simulink subsystem "Subsys_Conv_Ctrl_measurement_transformations"  (R2022b)
settings: Solver=VariableStepAuto  StartTime=0.0  StopTime=10.0  RelTol=1e-3
model mask{S_n=2e6, f_n=50, V_n_phph=690, V_n_grid_phph=20e3, V_n_dc=1380, meas_signals=0, meas_noise_filter=1, f_cutoff_lowpass=2500, posseq_calc=0, f_cutoff_posseq=20, prot_variant=1, v_dc_max=1.2, v_ac_max=1.1, t_ac_max=0.1, v_ac_maxmax=1.25, t_ac_maxmax=0.1, v_ac_min=0.8, t_ac_min=3, v_ac_minmin=0.45, t_ac_minmin=0.3, f_ac_max=51.5, t_f_ac_max=0.1, f_ac_maxmax=52.5, t_f_ac_maxmax=10, f_ac_min=47.5, t_f_ac_min=0.1, i_ac_max=1.25, T_s_ctrl=1e-3, T_s_PWM_meas=1e-4, datatype='double'}
  mask prompts: S_n "Nominal power [VA]"; f_n "Nominal frequency [Hz]"; V_n_phph "Nominal converter voltage (rms, phase-to-phase) [V]"; V_n_grid_phph "Nominal grid voltage (rms, phase-to-phase) [V]"; V_n_dc "Nominal DC-link voltage [V]"; meas_signals "Measured signals (0 = all signals (tDMSquared simulation), 1 = reduced signals (imperix hardware))"; meas_noise_filter "Low-pass to filter measurement noise (1 = enabled, 0 = disabled)"; f_cutoff_lowpass "Cutoff-frequency of low pass filter (measurement noise) [Hz]"; posseq_calc "Positive sequence calculation (0 = DDSRF, 1 = low pass filter)"; f_cutoff_posseq "Cutoff-frequency of low pass filter (positive sequence calculation) [Hz]"; prot_variant "Protection Variant (1 = hardware protection, 2 = tDMSquared warnings only, 3 = deactivated)"; v_dc_max "Maximum DC-link voltage [% nom. value]"; v_ac_max "Lower Maximum AC voltage [% nom. value]"; t_ac_max "Lower Maximum AC voltage timing [s]"; v_ac_maxmax "Upper Maximum AC voltage [% nom. value]"; t_ac_maxmax "Upper Maximum AC voltage timing [s]"; v_ac_min "Upper Minimum AC voltage [% nom. value]"; t_ac_min "Upper Minimum AC voltage timing [s]"; v_ac_minmin "Lower Minimum AC voltage [% nom. value]"; t_ac_minmin "Lower Minimum AC voltage timing [s]"; f_ac_max "Maximum AC frequency [Hz]"; t_f_ac_max "Maximum AC frequency timing [s]"; f_ac_maxmax "Upper Maximum AC frequency [Hz]"; t_f_ac_maxmax "Upper Maximum AC frequency timing [s]"; f_ac_min "Minimum AC frequency [Hz]"; t_f_ac_min "Minimum AC frequency timing [s]"; i_ac_max "Maximum AC current [% nom. value]"; T_s_ctrl "Controller sample time [s]"; T_s_PWM_meas "PWM and measurements sample time [s]"; datatype "Signal data type"
undefined symbols (not defined in the file): alpha_meas_LPF, alpha_posseq_LPF, den_HPF, num_HPF
libraries: eeTransforms x18
settings Model: Creator=winkens  LastModifiedBy=pc236admin
settings SolverCC: AlgebraicLoopSolver=TrustRegion
settings DebuggingCC: UnconnectedInputMsg=warning  UnconnectedOutputMsg=warning  UnconnectedLineMsg=warning  SFMachineParentedDataDiag=warning
settings ModelReferenceCC: EnableRefExpFcnMdlSchedulingChecks=on
settings RTWCC: DLArmComputeVersion=19.05

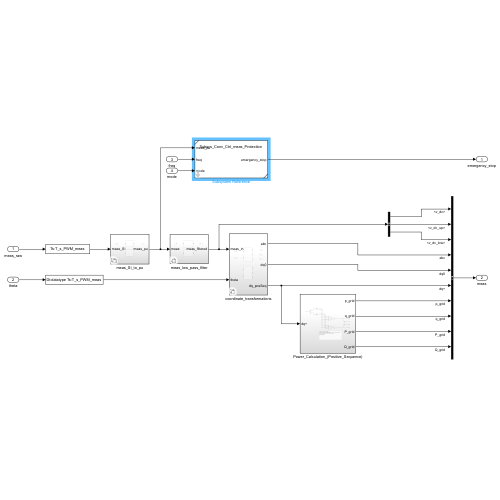
[thumbnail: Simulink's stored preview of the top-level diagram]
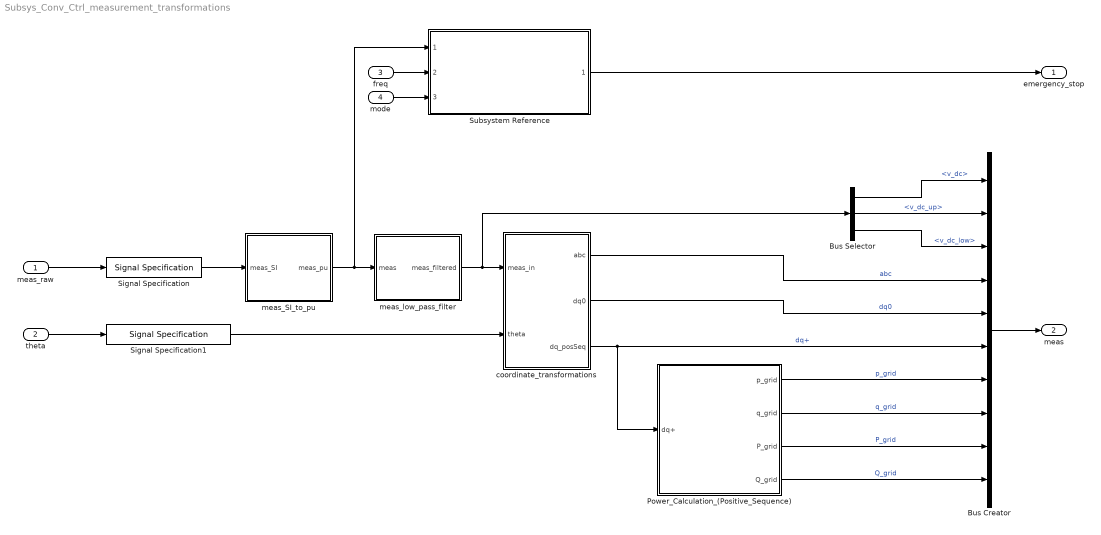
== system Subsys_Conv_Ctrl_measurement_transformations ==
  meas_raw : Inport
  theta : Inport  Port=2
  freq : Inport  Port=3
  mode : Inport  Port=4
  Bus Creator : BusCreator  Inputs=10
  Bus Selector : BusSelector  OutputSignals=v_dc,v_dc_up,v_dc_low
  Power_Calculation_(Positive_Sequence) : Subsystem
  Signal Specification : SignalSpecification  SampleTime=T_s_PWM_meas
  Signal Specification1 : SignalSpecification  OutDataTypeStr=datatype  SampleTime=T_s_PWM_meas
  Subsystem Reference : Subsystem  ReferencedSubsystem=Subsys_Conv_Ctrl_meas_Protection  prot_variant=prot_variant  f_n=f_n  meas_signals=meas_signals  v_n_dc=1  v_dc_max=v_dc_max  v_ac_max=v_ac_max  t_ac_max=t_ac_max  v_ac_maxmax=v_ac_maxmax  t_ac_maxmax=t_ac_maxmax  v_ac_min=v_ac_min  t_ac_min=t_ac_min  v_ac_minmin=v_ac_minmin  t_ac_minmin=t_ac_minmin  f_ac_max=f_ac_max  t_f_ac_max=t_f_ac_max  f_ac_maxmax=f_ac_maxmax  t_f_ac_maxmax=t_f_ac_maxmax  f_ac_min=f_ac_min  t_f_ac_min=t_f_ac_min  i_ac_max=i_ac_max  T_s=T_s_PWM_meas
  coordinate_transformations : Subsystem  Variant=on  VariantControl=Choice
  meas_SI_to_pu : Subsystem  Variant=on  VariantControl=Choice
  meas_low_pass_filter : Subsystem  Variant=on  VariantControl=Choice
  emergency_stop : Outport  OutDataTypeStr=boolean
  meas : Outport  Port=2
  wires:
  freq/1 -> Subsystem Reference/2
  theta/1 -> Signal Specification1/1
  meas_raw/1 -> Signal Specification/1
  meas_low_pass_filter/1(meas_filtered) -> Bus Selector/1, coordinate_transformations/1(meas_in)
  Bus Selector/1 -> Bus Creator/1  "<v_dc>"
  Power_Calculation_(Positive_Sequence)/1(p_grid) -> Bus Creator/7  "p_grid"
  Power_Calculation_(Positive_Sequence)/2(q_grid) -> Bus Creator/8  "q_grid"
  Power_Calculation_(Positive_Sequence)/3(P_grid) -> Bus Creator/9  "P_grid"
  Power_Calculation_(Positive_Sequence)/4(Q_grid) -> Bus Creator/10  "Q_grid"
  Bus Creator/1 -> meas/1
  Bus Selector/2 -> Bus Creator/2  "<v_dc_up>"
  Bus Selector/3 -> Bus Creator/3  "<v_dc_low>"
  Subsystem Reference/1 -> emergency_stop/1
  Signal Specification/1 -> meas_SI_to_pu/1(meas_SI)
  meas_SI_to_pu/1(meas_pu) -> meas_low_pass_filter/1(meas), Subsystem Reference/1
  Signal Specification1/1 -> coordinate_transformations/2(theta)
  coordinate_transformations/1(abc) -> Bus Creator/4  "abc"
  coordinate_transformations/2(dq0) -> Bus Creator/5  "dq0"
  coordinate_transformations/3(dq_posSeq) -> Bus Creator/6, Power_Calculation_(Positive_Sequence)/1(dq+)  "dq+"
  mode/1 -> Subsystem Reference/3

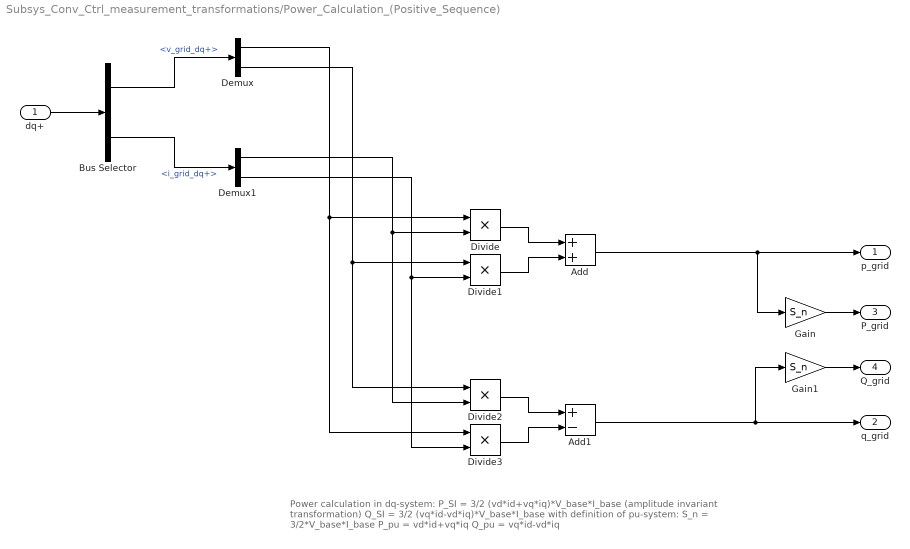
== system Subsys_Conv_Ctrl_measurement_transformations/Power_Calculation_(Positive_Sequence) ==
  note: Power calculation in dq-system:
      | P_SI = 3/2 (vd*id+vq*iq)*V_base*I_base (amplitude invariant transformation)
      | Q_SI = 3/2 (vq*id-vd*iq)*V_base*I_base
      | with definition of pu-system: S_n = 3/2*V_base*I_base
      | P_pu = vd*id+vq*iq
      | Q_pu = vq*id-vd*iq
  dq+ : Inport
  Add : Sum
  Add1 : Sum  Inputs=+-
  Bus Selector : BusSelector  OutputSignals=v_grid_dq+,i_grid_dq+
  Demux : Demux  Outputs=2
  Demux1 : Demux  Outputs=2
  Divide{,1..3} (4 alike) : Product  Inputs=**
  Gain : Gain  Gain=S_n
  Gain1 : Gain  Gain=S_n
  p_grid : Outport
  q_grid : Outport  Port=2
  P_grid : Outport  Port=3
  Q_grid : Outport  Port=4
  wires:
  Divide/1 -> Add/1
  Divide1/1 -> Add/2
  Divide2/1 -> Add1/1
  Divide3/1 -> Add1/2
  Add/1 -> Gain/1, p_grid/1
  Add1/1 -> Gain1/1, q_grid/1
  Demux/1 -> Divide3/1, Divide/1
  Demux1/1 -> Divide2/2, Divide/2
  Demux/2 -> Divide2/1, Divide1/1
  Demux1/2 -> Divide3/2, Divide1/2
  dq+/1 -> Bus Selector/1
  Bus Selector/1 -> Demux/1  "<v_grid_dq+>"
  Bus Selector/2 -> Demux1/1  "<i_grid_dq+>"
  Gain1/1 -> Q_grid/1
  Gain/1 -> P_grid/1

== system Subsys_Conv_Ctrl_measurement_transformations/coordinate_transformations ==
  meas_in : Inport
  theta : Inport  Port=2
  all_signals : Subsystem  VariantControl=(default)
  reduced_signals_imperix_hardware : Subsystem  VariantControl=meas_signals == 1
  abc : Outport
  dq0 : Outport  Port=2
  dq_posSeq : Outport  Port=3

== system Subsys_Conv_Ctrl_measurement_transformations/meas_SI_to_pu ==
  meas_SI : Inport
  all_signals : Subsystem  VariantControl=(default)
  reduced_signals_imperix_hardware : Subsystem  VariantControl=meas_signals == 1
  meas_pu : Outport

== system Subsys_Conv_Ctrl_measurement_transformations/meas_low_pass_filter ==
  meas : Inport
  low_pass_filter : Subsystem  Variant=on  VariantControl=meas_noise_filter > 0.5
  no_filter : Subsystem  Variant=on  VariantControl=(default)
  meas_filtered : Outport

== system Subsys_Conv_Ctrl_measurement_transformations/coordinate_transformations/all_signals ==
  meas_in : Inport
  theta : Inport  Port=2
  Positive_Sequence_(dq0->dq+) : Subsystem  Variant=on  VariantControl=Choice
  abc->dq0 : Subsystem
  abc : Outport
  dq0 : Outport  Port=2
  dq_posSeq : Outport  Port=3
  wires:
  meas_in/1 -> abc->dq0/2(meas)
  theta/1 -> abc->dq0/1(theta), Positive_Sequence_(dq0->dq+)/1(theta)
  abc->dq0/2(dq0) -> dq0/1, Positive_Sequence_(dq0->dq+)/2(dq0)
  abc->dq0/1(abc) -> abc/1
  Positive_Sequence_(dq0->dq+)/1(dq+) -> dq_posSeq/1

== system Subsys_Conv_Ctrl_measurement_transformations/coordinate_transformations/reduced_signals_imperix_hardware ==
  meas_in : Inport
  theta : Inport  Port=2
  Positive_Sequence_(dq0->dq+) : Subsystem  Variant=on  VariantControl=Choice
  abc->dq0 : Subsystem
  abc : Outport
  dq0 : Outport  Port=2
  dq_posSeq : Outport  Port=3
  wires:
  meas_in/1 -> abc->dq0/2(meas)
  theta/1 -> abc->dq0/1(theta), Positive_Sequence_(dq0->dq+)/1(theta)
  abc->dq0/2(dq0) -> dq0/1, Positive_Sequence_(dq0->dq+)/2(dq0)
  abc->dq0/1(abc) -> abc/1
  Positive_Sequence_(dq0->dq+)/1(dq+) -> dq_posSeq/1

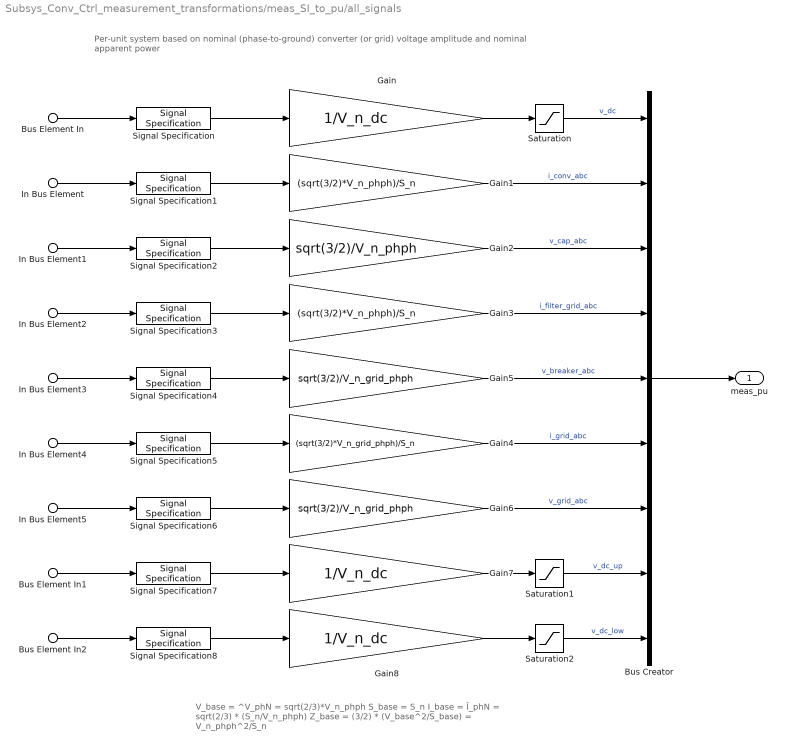
== system Subsys_Conv_Ctrl_measurement_transformations/meas_SI_to_pu/all_signals ==
  note: Per-unit system based on nominal (phase-to-ground) converter (or grid) voltage amplitude and nominal apparent power
  note: V_base = ^V_phN = sqrt(2/3)*V_n_phph
      | S_base = S_n
      | I_base = Î_phN = sqrt(2/3) * (S_n/V_n_phph)
      | Z_base = (3/2) * (V_base^2/S_base) = V_n_phph^2/S_n
  Bus Element In : Inport  PortName=meas_SI  Element=V_dc
  In Bus Element : Inport  PortName=meas_SI  Element=I_conv_abc
  In Bus Element1 : Inport  PortName=meas_SI  Element=V_cap_abc
  In Bus Element2 : Inport  PortName=meas_SI  Element=I_filter_grid_abc
  In Bus Element3 : Inport  PortName=meas_SI  Element=V_breaker_abc
  In Bus Element4 : Inport  PortName=meas_SI  Element=I_grid_abc
  In Bus Element5 : Inport  PortName=meas_SI  Element=V_grid_abc
  Bus Element In1 : Inport  PortName=meas_SI  Element=V_dc_up
  Bus Element In2 : Inport  PortName=meas_SI  Element=V_dc_low
  Bus Creator : BusCreator  Inputs=9
  Gain : Gain  Gain=1/V_n_dc
  Gain1 : Gain  Gain=(sqrt(3/2)*V_n_phph)/S_n
  Gain2 : Gain  Gain=sqrt(3/2)/V_n_phph
  Gain3 : Gain  Gain=(sqrt(3/2)*V_n_phph)/S_n
  Gain4 : Gain  Gain=(sqrt(3/2)*V_n_grid_phph)/S_n
  Gain5 : Gain  Gain=sqrt(3/2)/V_n_grid_phph
  Gain6 : Gain  Gain=sqrt(3/2)/V_n_grid_phph
  Gain7 : Gain  Gain=1/V_n_dc
  Gain8 : Gain  Gain=1/V_n_dc
  Saturation : Saturate  UpperLimit=inf  LowerLimit=0.01
  Saturation1 : Saturate  UpperLimit=inf  LowerLimit=0.01
  Saturation2 : Saturate  UpperLimit=inf  LowerLimit=0.01
  Signal Specification{,1..8} (9 alike) : SignalSpecification  OutDataTypeStr=datatype
  meas_pu : Outport
  wires:
  Bus Element In/1 -> Signal Specification/1
  In Bus Element/1 -> Signal Specification1/1
  In Bus Element1/1 -> Signal Specification2/1
  In Bus Element2/1 -> Signal Specification3/1
  In Bus Element3/1 -> Signal Specification4/1
  In Bus Element4/1 -> Signal Specification5/1
  In Bus Element5/1 -> Signal Specification6/1
  Gain/1 -> Saturation/1
  Gain1/1 -> Bus Creator/2  "i_conv_abc"
  Gain2/1 -> Bus Creator/3  "v_cap_abc"
  Gain3/1 -> Bus Creator/4  "i_filter_grid_abc"
  Gain5/1 -> Bus Creator/5  "v_breaker_abc"
  Gain4/1 -> Bus Creator/6  "i_grid_abc"
  Gain6/1 -> Bus Creator/7  "v_grid_abc"
  Bus Creator/1 -> meas_pu/1
  Bus Element In1/1 -> Signal Specification7/1
  Bus Element In2/1 -> Signal Specification8/1
  Gain7/1 -> Saturation1/1
  Gain8/1 -> Saturation2/1
  Saturation/1 -> Bus Creator/1  "v_dc"
  Saturation1/1 -> Bus Creator/8  "v_dc_up"
  Saturation2/1 -> Bus Creator/9  "v_dc_low"
  Signal Specification/1 -> Gain/1
  Signal Specification1/1 -> Gain1/1
  Signal Specification2/1 -> Gain2/1
  Signal Specification3/1 -> Gain3/1
  Signal Specification4/1 -> Gain5/1
  Signal Specification5/1 -> Gain4/1
  Signal Specification6/1 -> Gain6/1
  Signal Specification7/1 -> Gain7/1
  Signal Specification8/1 -> Gain8/1

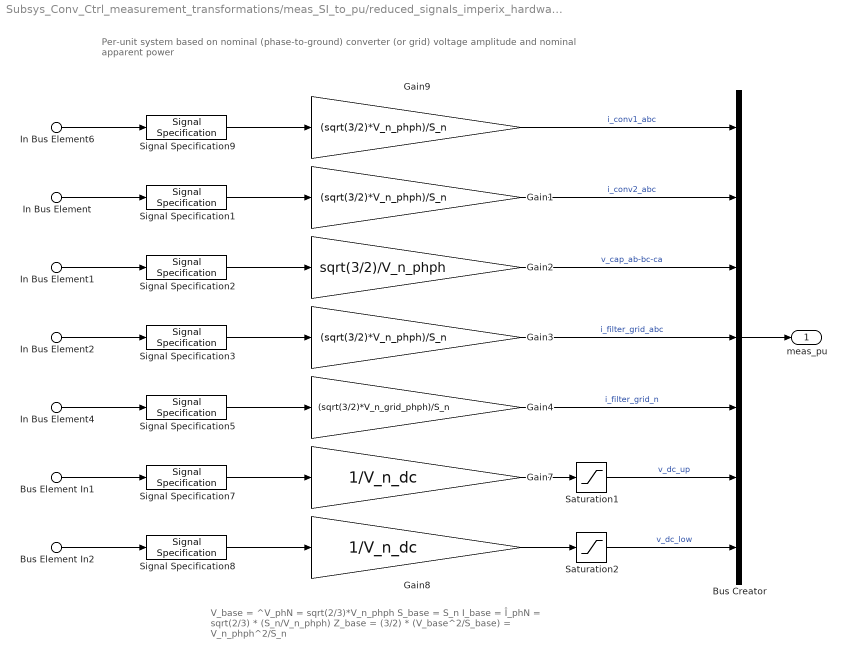
== system Subsys_Conv_Ctrl_measurement_transformations/meas_SI_to_pu/reduced_signals_imperix_hardware ==
  note: Per-unit system based on nominal (phase-to-ground) converter (or grid) voltage amplitude and nominal apparent power
  note: V_base = ^V_phN = sqrt(2/3)*V_n_phph
      | S_base = S_n
      | I_base = Î_phN = sqrt(2/3) * (S_n/V_n_phph)
      | Z_base = (3/2) * (V_base^2/S_base) = V_n_phph^2/S_n
  In Bus Element : Inport  PortName=meas_SI  Element=I_conv2_abc
  In Bus Element1 : Inport  PortName=meas_SI  Element=V_cap_ab-bc-ca
  In Bus Element2 : Inport  PortName=meas_SI  Element=I_filter_grid_abc
  In Bus Element4 : Inport  PortName=meas_SI  Element=I_filter_grid_n
  Bus Element In1 : Inport  PortName=meas_SI  Element=V_dc_up
  Bus Element In2 : Inport  PortName=meas_SI  Element=V_dc_low
  In Bus Element6 : Inport  PortName=meas_SI  Element=I_conv1_abc
  Bus Creator : BusCreator  Inputs=7
  Gain1 : Gain  Gain=(sqrt(3/2)*V_n_phph)/S_n
  Gain2 : Gain  Gain=sqrt(3/2)/V_n_phph
  Gain3 : Gain  Gain=(sqrt(3/2)*V_n_phph)/S_n
  Gain4 : Gain  Gain=(sqrt(3/2)*V_n_grid_phph)/S_n
  Gain7 : Gain  Gain=1/V_n_dc
  Gain8 : Gain  Gain=1/V_n_dc
  Gain9 : Gain  Gain=(sqrt(3/2)*V_n_phph)/S_n
  Saturation1 : Saturate  UpperLimit=inf  LowerLimit=0.01
  Saturation2 : Saturate  UpperLimit=inf  LowerLimit=0.01
  Signal Specification{1..3,5,7..9} (7 alike) : SignalSpecification  OutDataTypeStr=datatype
  meas_pu : Outport
  wires:
  In Bus Element/1 -> Signal Specification1/1
  In Bus Element1/1 -> Signal Specification2/1
  In Bus Element2/1 -> Signal Specification3/1
  In Bus Element4/1 -> Signal Specification5/1
  Gain1/1 -> Bus Creator/2  "i_conv2_abc"
  Gain2/1 -> Bus Creator/3  "v_cap_ab-bc-ca"
  Gain3/1 -> Bus Creator/4  "i_filter_grid_abc"
  Gain4/1 -> Bus Creator/5  "i_filter_grid_n"
  Bus Creator/1 -> meas_pu/1
  Bus Element In1/1 -> Signal Specification7/1
  Bus Element In2/1 -> Signal Specification8/1
  Gain7/1 -> Saturation1/1
  Gain8/1 -> Saturation2/1
  Saturation1/1 -> Bus Creator/6  "v_dc_up"
  Saturation2/1 -> Bus Creator/7  "v_dc_low"
  Signal Specification1/1 -> Gain1/1
  Signal Specification2/1 -> Gain2/1
  Signal Specification3/1 -> Gain3/1
  Signal Specification5/1 -> Gain4/1
  Signal Specification7/1 -> Gain7/1
  Signal Specification8/1 -> Gain8/1
  Signal Specification9/1 -> Gain9/1
  Gain9/1 -> Bus Creator/1  "i_conv1_abc"
  In Bus Element6/1 -> Signal Specification9/1

== system Subsys_Conv_Ctrl_measurement_transformations/meas_low_pass_filter/low_pass_filter ==
  meas : Inport
  all_signals : Subsystem  VariantControl=(default)
  reduced_signals_imperix_hardware : Subsystem  VariantControl=meas_signals == 1
  meas_filtered : Outport

== system Subsys_Conv_Ctrl_measurement_transformations/meas_low_pass_filter/no_filter ==
  meas : Inport
  all_signals : Subsystem  VariantControl=(default)
  reduced_signals_imperix_hardware : Subsystem  VariantControl=meas_signals == 1
  meas_filtered : Outport

== system Subsys_Conv_Ctrl_measurement_transformations/coordinate_transformations/all_signals/Positive_Sequence_(dq0->dq+) ==
  theta : Inport
  dq0 : Inport  Port=2
  DDSRF : Subsystem  VariantControl=posseq_calc == 0
  LPF : Subsystem  VariantControl=posseq_calc == 1
  dq+ : Outport

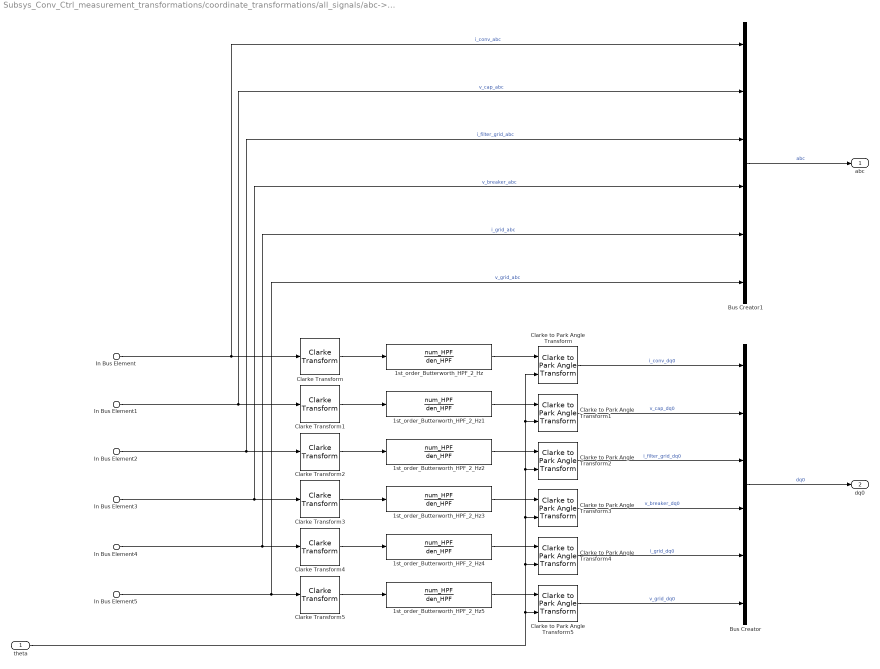
== system Subsys_Conv_Ctrl_measurement_transformations/coordinate_transformations/all_signals/abc->dq0 ==
  theta : Inport
  In Bus Element : Inport  Port=2  PortName=meas  Element=i_conv_abc
  In Bus Element1 : Inport  Port=2  PortName=meas  Element=v_cap_abc
  In Bus Element2 : Inport  Port=2  PortName=meas  Element=i_filter_grid_abc
  In Bus Element3 : Inport  Port=2  PortName=meas  Element=v_breaker_abc
  In Bus Element4 : Inport  Port=2  PortName=meas  Element=i_grid_abc
  In Bus Element5 : Inport  Port=2  PortName=meas  Element=v_grid_abc
  1st_order_Butterworth_HPF_2_Hz{,1..5} (6 alike) : DiscreteFilter  Numerator=num_HPF  Denominator=den_HPF  SampleTime=T_s_PWM_meas
  Bus Creator : BusCreator  Inputs=6
  Bus Creator1 : BusCreator  Inputs=6
  Clarke Transform{,1..5} (6 alike) : eeTransforms/Clarke Transform  PowerInvariant=off
  Clarke to Park Angle Transform{,1..5} (6 alike) : eeTransforms/Clarke to Park Angle Transform  AxisAlignment=D-axis
  abc : Outport
  dq0 : Outport  Port=2
  wires:
  Clarke to Park Angle Transform4/1 -> Bus Creator/5  "i_grid_dq0"
  Clarke to Park Angle Transform2/1 -> Bus Creator/3  "i_filter_grid_dq0"
  In Bus Element2/1 -> Clarke Transform2/1, Bus Creator1/3  "i_filter_grid_abc"
  In Bus Element4/1 -> Clarke Transform4/1, Bus Creator1/5  "i_grid_abc"
  In Bus Element1/1 -> Clarke Transform1/1, Bus Creator1/2  "v_cap_abc"
  Clarke to Park Angle Transform1/1 -> Bus Creator/2  "v_cap_dq0"
  Clarke to Park Angle Transform/1 -> Bus Creator/1  "i_conv_dq0"
  In Bus Element/1 -> Clarke Transform/1, Bus Creator1/1  "i_conv_abc"
  In Bus Element3/1 -> Clarke Transform3/1, Bus Creator1/4  "v_breaker_abc"
  Bus Creator/1 -> dq0/1  "dq0"
  In Bus Element5/1 -> Clarke Transform5/1, Bus Creator1/6  "v_grid_abc"
  Bus Creator1/1 -> abc/1  "abc"
  Clarke to Park Angle Transform3/1 -> Bus Creator/4  "v_breaker_dq0"
  Clarke Transform/1 -> 1st_order_Butterworth_HPF_2_Hz/1
  Clarke to Park Angle Transform5/1 -> Bus Creator/6  "v_grid_dq0"
  theta/1 -> Clarke to Park Angle Transform/2, Clarke to Park Angle Transform1/2, Clarke to Park Angle Transform2/2, Clarke to Park Angle Transform3/2, Clarke to Park Angle Transform4/2, Clarke to Park Angle Transform5/2
  Clarke Transform1/1 -> 1st_order_Butterworth_HPF_2_Hz1/1
  Clarke Transform2/1 -> 1st_order_Butterworth_HPF_2_Hz2/1
  Clarke Transform3/1 -> 1st_order_Butterworth_HPF_2_Hz3/1
  Clarke Transform4/1 -> 1st_order_Butterworth_HPF_2_Hz4/1
  Clarke Transform5/1 -> 1st_order_Butterworth_HPF_2_Hz5/1
  1st_order_Butterworth_HPF_2_Hz/1 -> Clarke to Park Angle Transform/1
  1st_order_Butterworth_HPF_2_Hz1/1 -> Clarke to Park Angle Transform1/1
  1st_order_Butterworth_HPF_2_Hz2/1 -> Clarke to Park Angle Transform2/1
  1st_order_Butterworth_HPF_2_Hz3/1 -> Clarke to Park Angle Transform3/1
  1st_order_Butterworth_HPF_2_Hz4/1 -> Clarke to Park Angle Transform4/1
  1st_order_Butterworth_HPF_2_Hz5/1 -> Clarke to Park Angle Transform5/1

== system Subsys_Conv_Ctrl_measurement_transformations/coordinate_transformations/reduced_signals_imperix_hardware/Positive_Sequence_(dq0->dq+) ==
  theta : Inport
  dq0 : Inport  Port=2
  DDSRF : Subsystem  VariantControl=posseq_calc == 0
  LPF : Subsystem  VariantControl=posseq_calc == 1
  dq+ : Outport

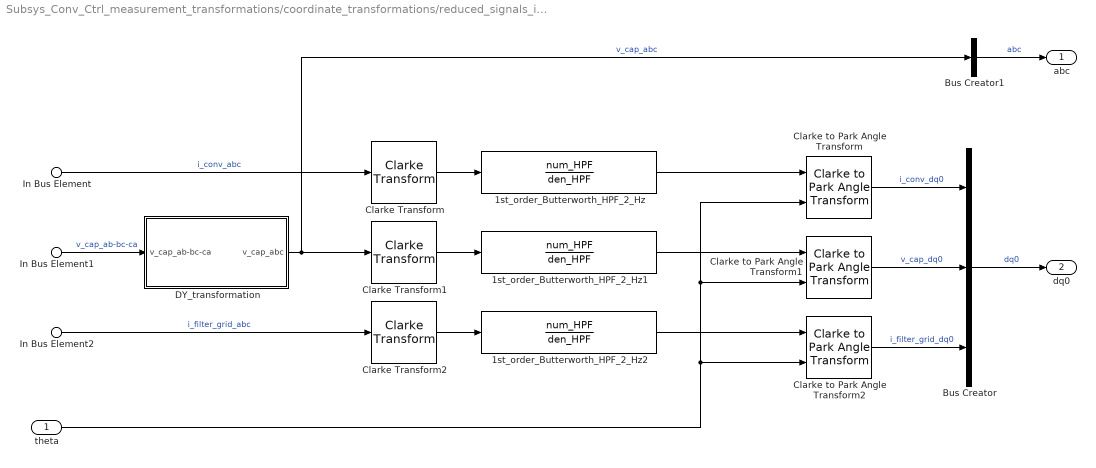
== system Subsys_Conv_Ctrl_measurement_transformations/coordinate_transformations/reduced_signals_imperix_hardware/abc->dq0 ==
  theta : Inport
  In Bus Element : Inport  Port=2  PortName=meas  Element=i_conv_abc
  In Bus Element1 : Inport  Port=2  PortName=meas  Element=v_cap_ab-bc-ca
  In Bus Element2 : Inport  Port=2  PortName=meas  Element=i_filter_grid_abc
  1st_order_Butterworth_HPF_2_Hz : DiscreteFilter  Numerator=num_HPF  Denominator=den_HPF  SampleTime=T_s_PWM_meas
  1st_order_Butterworth_HPF_2_Hz1 : DiscreteFilter  Numerator=num_HPF  Denominator=den_HPF  SampleTime=T_s_PWM_meas
  1st_order_Butterworth_HPF_2_Hz2 : DiscreteFilter  Numerator=num_HPF  Denominator=den_HPF  SampleTime=T_s_PWM_meas
  Bus Creator : BusCreator  Inputs=3
  Bus Creator1 : BusCreator  Inputs=1
  Clarke Transform : eeTransforms/Clarke Transform  PowerInvariant=off
  Clarke Transform1 : eeTransforms/Clarke Transform  PowerInvariant=off
  Clarke Transform2 : eeTransforms/Clarke Transform  PowerInvariant=off
  Clarke to Park Angle Transform : eeTransforms/Clarke to Park Angle Transform  AxisAlignment=D-axis
  Clarke to Park Angle Transform1 : eeTransforms/Clarke to Park Angle Transform  AxisAlignment=D-axis
  Clarke to Park Angle Transform2 : eeTransforms/Clarke to Park Angle Transform  AxisAlignment=D-axis
  DY_transformation : Subsystem
  abc : Outport
  dq0 : Outport  Port=2
  wires:
  Clarke to Park Angle Transform2/1 -> Bus Creator/3  "i_filter_grid_dq0"
  In Bus Element2/1 -> Clarke Transform2/1  "i_filter_grid_abc"
  In Bus Element1/1 -> DY_transformation/1(v_cap_ab-bc-ca)  "v_cap_ab-bc-ca"
  Clarke to Park Angle Transform/1 -> Bus Creator/1  "i_conv_dq0"
  In Bus Element/1 -> Clarke Transform/1  "i_conv_abc"
  Bus Creator/1 -> dq0/1  "dq0"
  Clarke to Park Angle Transform1/1 -> Bus Creator/2  "v_cap_dq0"
  Bus Creator1/1 -> abc/1  "abc"
  Clarke Transform2/1 -> 1st_order_Butterworth_HPF_2_Hz2/1
  Clarke Transform1/1 -> 1st_order_Butterworth_HPF_2_Hz1/1
  Clarke Transform/1 -> 1st_order_Butterworth_HPF_2_Hz/1
  1st_order_Butterworth_HPF_2_Hz/1 -> Clarke to Park Angle Transform/1
  1st_order_Butterworth_HPF_2_Hz1/1 -> Clarke to Park Angle Transform1/1
  1st_order_Butterworth_HPF_2_Hz2/1 -> Clarke to Park Angle Transform2/1
  theta/1 -> Clarke to Park Angle Transform2/2, Clarke to Park Angle Transform1/2, Clarke to Park Angle Transform/2
  DY_transformation/1(v_cap_abc) -> Clarke Transform1/1, Bus Creator1/1  "v_cap_abc"

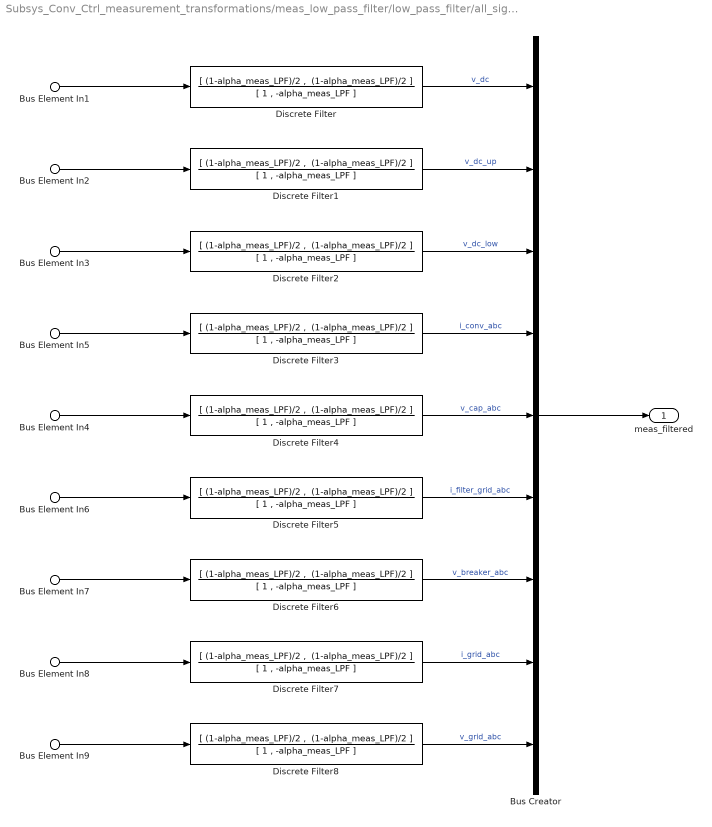
== system Subsys_Conv_Ctrl_measurement_transformations/meas_low_pass_filter/low_pass_filter/all_signals ==
  Bus Element In4 : Inport  PortName=meas  Element=v_cap_abc
  Bus Element In1 : Inport  PortName=meas  Element=v_dc
  Bus Element In2 : Inport  PortName=meas  Element=v_dc_up
  Bus Element In3 : Inport  PortName=meas  Element=v_dc_low
  Bus Element In5 : Inport  PortName=meas  Element=i_conv_abc
  Bus Element In6 : Inport  PortName=meas  Element=i_filter_grid_abc
  Bus Element In7 : Inport  PortName=meas  Element=v_breaker_abc
  Bus Element In8 : Inport  PortName=meas  Element=i_grid_abc
  Bus Element In9 : Inport  PortName=meas  Element=v_grid_abc
  Bus Creator : BusCreator  Inputs=9
  Discrete Filter{,1..8} (9 alike) : DiscreteFilter  Numerator="[ (1-alpha_meas_LPF)/2 ,  (1-alpha_meas_LPF)/2 ]"  Denominator=[ 1 , -alpha_meas_LPF ]  SampleTime=T_s_PWM_meas
  meas_filtered : Outport
  wires:
  Bus Element In1/1 -> Discrete Filter/1
  Bus Element In5/1 -> Discrete Filter3/1
  Bus Element In4/1 -> Discrete Filter4/1
  Bus Element In6/1 -> Discrete Filter5/1
  Bus Element In7/1 -> Discrete Filter6/1
  Bus Element In8/1 -> Discrete Filter7/1
  Discrete Filter6/1 -> Bus Creator/7  "v_breaker_abc"
  Discrete Filter5/1 -> Bus Creator/6  "i_filter_grid_abc"
  Discrete Filter4/1 -> Bus Creator/5  "v_cap_abc"
  Discrete Filter3/1 -> Bus Creator/4  "i_conv_abc"
  Discrete Filter/1 -> Bus Creator/1  "v_dc"
  Discrete Filter7/1 -> Bus Creator/8  "i_grid_abc"
  Bus Element In9/1 -> Discrete Filter8/1
  Discrete Filter8/1 -> Bus Creator/9  "v_grid_abc"
  Bus Creator/1 -> meas_filtered/1
  Bus Element In3/1 -> Discrete Filter2/1
  Bus Element In2/1 -> Discrete Filter1/1
  Discrete Filter1/1 -> Bus Creator/2  "v_dc_up"
  Discrete Filter2/1 -> Bus Creator/3  "v_dc_low"

== system Subsys_Conv_Ctrl_measurement_transformations/meas_low_pass_filter/low_pass_filter/reduced_signals_imperix_hardware ==
  Bus Element In : Inport  PortName=meas  Element=v_dc_up
  Bus Element In1 : Inport  PortName=meas  Element=v_dc_low
  Bus Element In2 : Inport  PortName=meas  Element=i_conv1_abc
  Bus Element In3 : Inport  PortName=meas  Element=i_conv2_abc
  Bus Element In4 : Inport  PortName=meas  Element=v_cap_ab-bc-ca
  Bus Element In5 : Inport  PortName=meas  Element=i_filter_grid_abc
  Add : Sum
  Add1 : Sum
  Bus Creator : BusCreator  Inputs=6
  Discrete Filter{1..5} (5 alike) : DiscreteFilter  Numerator="[ (1-alpha_meas_LPF)/2 ,  (1-alpha_meas_LPF)/2 ]"  Denominator=[ 1 , -alpha_meas_LPF ]  SampleTime=T_s_PWM_meas
  meas_filtered : Outport
  wires:
  Add1/1 -> Discrete Filter3/1
  Bus Element In4/1 -> Discrete Filter4/1
  Bus Element In5/1 -> Discrete Filter5/1
  Discrete Filter5/1 -> Bus Creator/6  "i_filter_grid_abc"
  Discrete Filter4/1 -> Bus Creator/5  "v_cap_ab-bc-ca"
  Discrete Filter3/1 -> Bus Creator/4  "i_conv_abc"
  Bus Creator/1 -> meas_filtered/1
  Bus Element In1/1 -> Discrete Filter2/1
  Bus Element In/1 -> Discrete Filter1/1
  Discrete Filter1/1 -> Add/2, Bus Creator/1  "v_dc_up"
  Discrete Filter2/1 -> Add/1, Bus Creator/2  "v_dc_low"
  Add/1 -> Bus Creator/3  "v_dc"
  Bus Element In3/1 -> Add1/2
  Bus Element In2/1 -> Add1/1

== system Subsys_Conv_Ctrl_measurement_transformations/meas_low_pass_filter/no_filter/all_signals ==
  meas : Inport
  meas_filtered : Outport
  wires:
  meas/1 -> meas_filtered/1

== system Subsys_Conv_Ctrl_measurement_transformations/meas_low_pass_filter/no_filter/reduced_signals_imperix_hardware ==
  Bus Element In : Inport  PortName=meas  Element=v_dc_up
  Bus Element In1 : Inport  PortName=meas  Element=v_dc_low
  Bus Element In2 : Inport  PortName=meas  Element=i_conv1_abc
  Bus Element In3 : Inport  PortName=meas  Element=i_conv2_abc
  Bus Element In4 : Inport  PortName=meas  Element=v_cap_ab-bc-ca
  Bus Element In5 : Inport  PortName=meas  Element=i_filter_grid_abc
  Add : Sum
  Add1 : Sum
  Bus Creator : BusCreator  Inputs=6
  meas_filtered : Outport
  wires:
  Add1/1 -> Bus Creator/4  "i_conv_abc"
  Bus Element In5/1 -> Bus Creator/6  "i_filter_grid_abc"
  Bus Element In/1 -> Add/2, Bus Creator/1  "v_dc_up"
  Add/1 -> Bus Creator/3  "v_dc"
  Bus Element In3/1 -> Add1/2
  Bus Element In4/1 -> Bus Creator/5  "v_cap_ab-bc-ca"
  Bus Element In2/1 -> Add1/1
  Bus Element In1/1 -> Add/1, Bus Creator/2  "v_dc_low"
  Bus Creator/1 -> meas_filtered/1

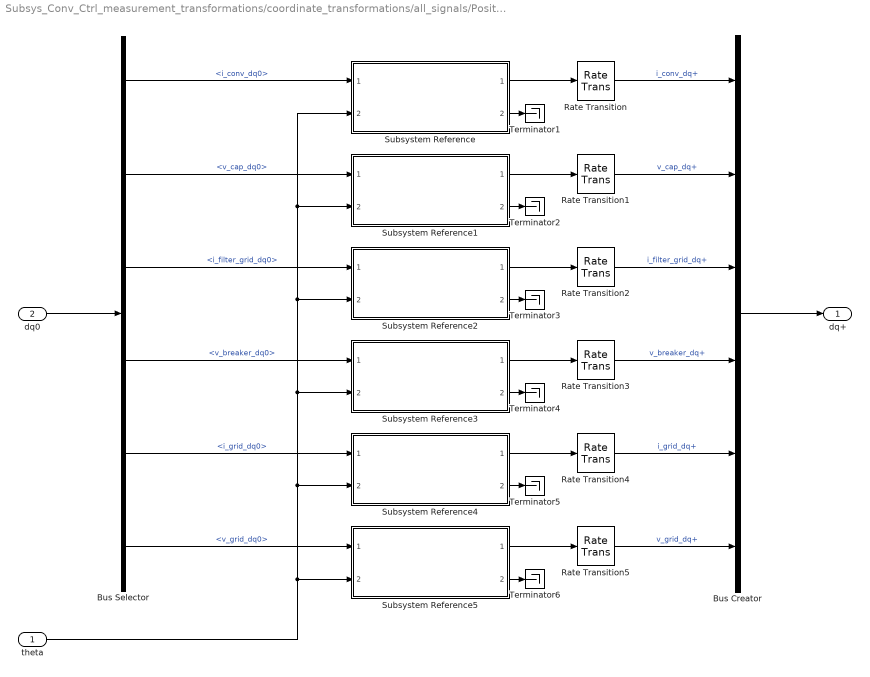
== system Subsys_Conv_Ctrl_measurement_transformations/coordinate_transformations/all_signals/Positive_Sequence_(dq0->dq+)/DDSRF ==
  theta : Inport
  dq0 : Inport  Port=2
  Bus Creator : BusCreator  Inputs=6
  Bus Selector : BusSelector  OutputSignals=i_conv_dq0,v_cap_dq0,i_filter_grid_dq0,v_breaker_dq0,i_grid_dq0,v_grid_dq0
  Rate Transition{,1..5} (6 alike) : RateTransition  Deterministic=off  OutPortSampleTime=T_s_ctrl
  Subsystem Reference{,1..5} (6 alike) : Subsystem  ReferencedSubsystem=DDSRF  f_n=f_n  T_s=T_s_PWM_meas
  Terminator{1..6} (6 alike) : Terminator
  dq+ : Outport
  wires:
  dq0/1 -> Bus Selector/1
  Bus Selector/1 -> Subsystem Reference/1  "<i_conv_dq0>"
  Bus Selector/2 -> Subsystem Reference1/1  "<v_cap_dq0>"
  Bus Selector/3 -> Subsystem Reference2/1  "<i_filter_grid_dq0>"
  Bus Selector/4 -> Subsystem Reference3/1  "<v_breaker_dq0>"
  Bus Selector/5 -> Subsystem Reference4/1  "<i_grid_dq0>"
  Bus Selector/6 -> Subsystem Reference5/1  "<v_grid_dq0>"
  Subsystem Reference/1 -> Rate Transition/1
  Subsystem Reference1/1 -> Rate Transition1/1
  Subsystem Reference2/1 -> Rate Transition2/1
  Subsystem Reference3/1 -> Rate Transition3/1
  Subsystem Reference4/1 -> Rate Transition4/1
  Subsystem Reference5/1 -> Rate Transition5/1
  Bus Creator/1 -> dq+/1
  Rate Transition/1 -> Bus Creator/1  "i_conv_dq+"
  Rate Transition1/1 -> Bus Creator/2  "v_cap_dq+"
  Rate Transition2/1 -> Bus Creator/3  "i_filter_grid_dq+"
  Rate Transition3/1 -> Bus Creator/4  "v_breaker_dq+"
  Rate Transition4/1 -> Bus Creator/5  "i_grid_dq+"
  Rate Transition5/1 -> Bus Creator/6  "v_grid_dq+"
  theta/1 -> Subsystem Reference5/2, Subsystem Reference4/2, Subsystem Reference3/2, Subsystem Reference2/2, Subsystem Reference1/2, Subsystem Reference/2
  Subsystem Reference/2 -> Terminator1/1
  Subsystem Reference1/2 -> Terminator2/1
  Subsystem Reference2/2 -> Terminator3/1
  Subsystem Reference3/2 -> Terminator4/1
  Subsystem Reference4/2 -> Terminator5/1
  Subsystem Reference5/2 -> Terminator6/1

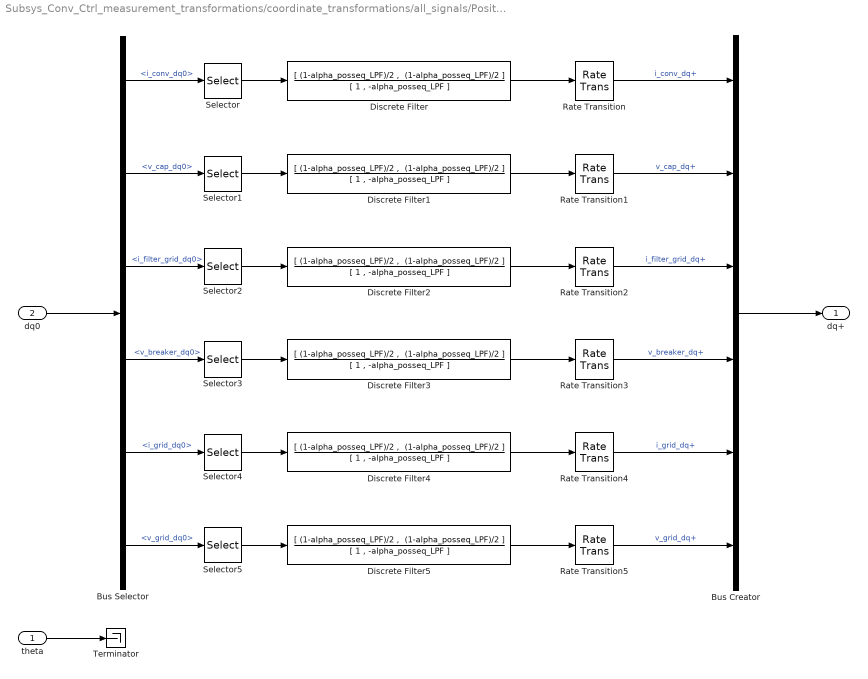
== system Subsys_Conv_Ctrl_measurement_transformations/coordinate_transformations/all_signals/Positive_Sequence_(dq0->dq+)/LPF ==
  theta : Inport
  dq0 : Inport  Port=2
  Bus Creator : BusCreator  Inputs=6
  Bus Selector : BusSelector  OutputSignals=i_conv_dq0,v_cap_dq0,i_filter_grid_dq0,v_breaker_dq0,i_grid_dq0,v_grid_dq0
  Discrete Filter{,1..5} (6 alike) : DiscreteFilter  Numerator="[ (1-alpha_posseq_LPF)/2 ,  (1-alpha_posseq_LPF)/2 ]"  Denominator=[ 1 , -alpha_posseq_LPF ]  SampleTime=T_s_PWM_meas
  Rate Transition{,1..5} (6 alike) : RateTransition  Deterministic=off  OutPortSampleTime=T_s_ctrl
  Selector{,1..5} (6 alike) : Selector  InputPortWidth=3  IndexOptions=Index vector (dialog)  Indices=[1 2]  OutputSizes=1
  Terminator : Terminator
  dq+ : Outport
  wires:
  dq0/1 -> Bus Selector/1
  Bus Selector/1 -> Selector/1  "<i_conv_dq0>"
  Bus Selector/2 -> Selector1/1  "<v_cap_dq0>"
  Bus Selector/3 -> Selector2/1  "<i_filter_grid_dq0>"
  Bus Selector/4 -> Selector3/1  "<v_breaker_dq0>"
  Bus Selector/5 -> Selector4/1  "<i_grid_dq0>"
  Bus Selector/6 -> Selector5/1  "<v_grid_dq0>"
  Discrete Filter/1 -> Rate Transition/1
  Discrete Filter1/1 -> Rate Transition1/1
  Discrete Filter2/1 -> Rate Transition2/1
  Discrete Filter3/1 -> Rate Transition3/1
  Discrete Filter4/1 -> Rate Transition4/1
  Discrete Filter5/1 -> Rate Transition5/1
  Bus Creator/1 -> dq+/1
  Selector/1 -> Discrete Filter/1
  Selector1/1 -> Discrete Filter1/1
  Selector2/1 -> Discrete Filter2/1
  Selector3/1 -> Discrete Filter3/1
  Selector4/1 -> Discrete Filter4/1
  Selector5/1 -> Discrete Filter5/1
  Rate Transition/1 -> Bus Creator/1  "i_conv_dq+"
  Rate Transition1/1 -> Bus Creator/2  "v_cap_dq+"
  Rate Transition2/1 -> Bus Creator/3  "i_filter_grid_dq+"
  Rate Transition3/1 -> Bus Creator/4  "v_breaker_dq+"
  Rate Transition4/1 -> Bus Creator/5  "i_grid_dq+"
  Rate Transition5/1 -> Bus Creator/6  "v_grid_dq+"
  theta/1 -> Terminator/1

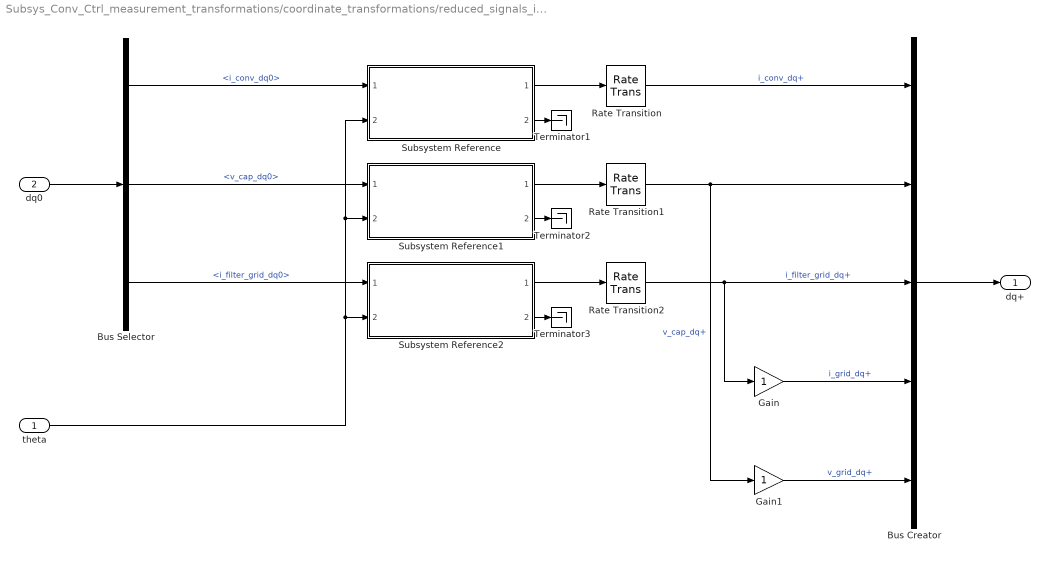
== system Subsys_Conv_Ctrl_measurement_transformations/coordinate_transformations/reduced_signals_imperix_hardware/Positive_Sequence_(dq0->dq+)/DDSRF ==
  theta : Inport
  dq0 : Inport  Port=2
  Bus Creator : BusCreator  Inputs=5
  Bus Selector : BusSelector  OutputSignals=i_conv_dq0,v_cap_dq0,i_filter_grid_dq0
  Gain : Gain
  Gain1 : Gain
  Rate Transition : RateTransition  Deterministic=off  OutPortSampleTime=T_s_ctrl
  Rate Transition1 : RateTransition  Deterministic=off  OutPortSampleTime=T_s_ctrl
  Rate Transition2 : RateTransition  Deterministic=off  OutPortSampleTime=T_s_ctrl
  Subsystem Reference : Subsystem  ReferencedSubsystem=DDSRF  f_n=f_n  T_s=T_s_PWM_meas
  Subsystem Reference1 : Subsystem  ReferencedSubsystem=DDSRF  f_n=f_n  T_s=T_s_PWM_meas
  Subsystem Reference2 : Subsystem  ReferencedSubsystem=DDSRF  f_n=f_n  T_s=T_s_PWM_meas
  Terminator1 : Terminator
  Terminator2 : Terminator
  Terminator3 : Terminator
  dq+ : Outport
  wires:
  dq0/1 -> Bus Selector/1
  Bus Selector/1 -> Subsystem Reference/1  "<i_conv_dq0>"
  Bus Selector/2 -> Subsystem Reference1/1  "<v_cap_dq0>"
  Bus Selector/3 -> Subsystem Reference2/1  "<i_filter_grid_dq0>"
  Subsystem Reference/1 -> Rate Transition/1
  Subsystem Reference1/1 -> Rate Transition1/1
  Subsystem Reference2/1 -> Rate Transition2/1
  Bus Creator/1 -> dq+/1
  Rate Transition/1 -> Bus Creator/1  "i_conv_dq+"
  Rate Transition1/1 -> Gain1/1, Bus Creator/2  "v_cap_dq+"
  Rate Transition2/1 -> Gain/1, Bus Creator/3  "i_filter_grid_dq+"
  Gain/1 -> Bus Creator/4  "i_grid_dq+"
  Gain1/1 -> Bus Creator/5  "v_grid_dq+"
  Subsystem Reference/2 -> Terminator1/1
  Subsystem Reference1/2 -> Terminator2/1
  Subsystem Reference2/2 -> Terminator3/1
  theta/1 -> Subsystem Reference2/2, Subsystem Reference1/2, Subsystem Reference/2

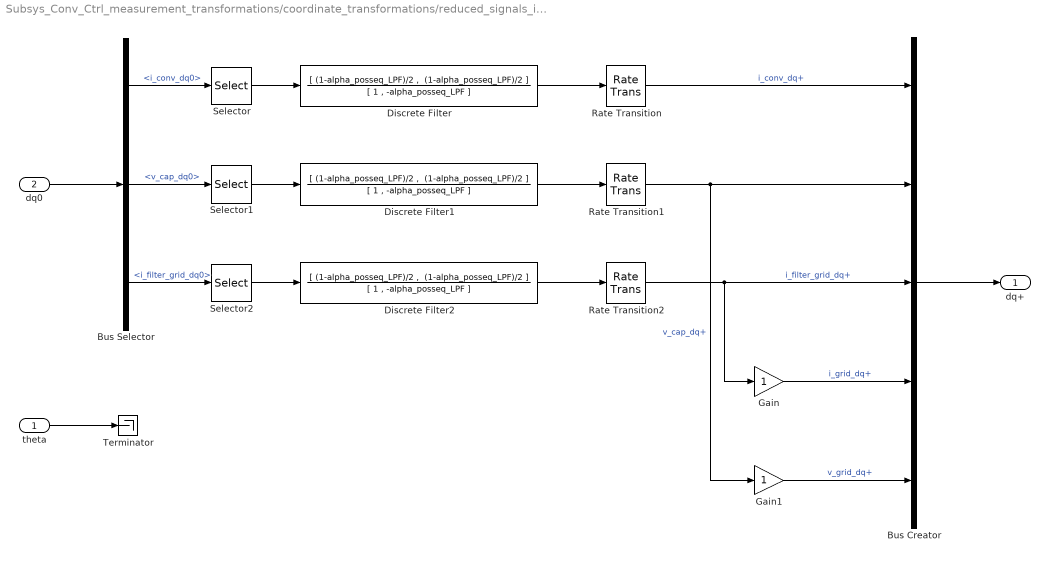
== system Subsys_Conv_Ctrl_measurement_transformations/coordinate_transformations/reduced_signals_imperix_hardware/Positive_Sequence_(dq0->dq+)/LPF ==
  theta : Inport
  dq0 : Inport  Port=2
  Bus Creator : BusCreator  Inputs=5
  Bus Selector : BusSelector  OutputSignals=i_conv_dq0,v_cap_dq0,i_filter_grid_dq0
  Discrete Filter : DiscreteFilter  Numerator="[ (1-alpha_posseq_LPF)/2 ,  (1-alpha_posseq_LPF)/2 ]"  Denominator=[ 1 , -alpha_posseq_LPF ]  SampleTime=T_s_PWM_meas
  Discrete Filter1 : DiscreteFilter  Numerator="[ (1-alpha_posseq_LPF)/2 ,  (1-alpha_posseq_LPF)/2 ]"  Denominator=[ 1 , -alpha_posseq_LPF ]  SampleTime=T_s_PWM_meas
  Discrete Filter2 : DiscreteFilter  Numerator="[ (1-alpha_posseq_LPF)/2 ,  (1-alpha_posseq_LPF)/2 ]"  Denominator=[ 1 , -alpha_posseq_LPF ]  SampleTime=T_s_PWM_meas
  Gain : Gain
  Gain1 : Gain
  Rate Transition : RateTransition  Deterministic=off  OutPortSampleTime=T_s_ctrl
  Rate Transition1 : RateTransition  Deterministic=off  OutPortSampleTime=T_s_ctrl
  Rate Transition2 : RateTransition  Deterministic=off  OutPortSampleTime=T_s_ctrl
  Selector : Selector  InputPortWidth=3  IndexOptions=Index vector (dialog)  Indices=[1 2]  OutputSizes=1
  Selector1 : Selector  InputPortWidth=3  IndexOptions=Index vector (dialog)  Indices=[1 2]  OutputSizes=1
  Selector2 : Selector  InputPortWidth=3  IndexOptions=Index vector (dialog)  Indices=[1 2]  OutputSizes=1
  Terminator : Terminator
  dq+ : Outport
  wires:
  dq0/1 -> Bus Selector/1
  Bus Selector/1 -> Selector/1  "<i_conv_dq0>"
  Bus Selector/2 -> Selector1/1  "<v_cap_dq0>"
  Bus Selector/3 -> Selector2/1  "<i_filter_grid_dq0>"
  Discrete Filter/1 -> Rate Transition/1
  Discrete Filter1/1 -> Rate Transition1/1
  Discrete Filter2/1 -> Rate Transition2/1
  Bus Creator/1 -> dq+/1
  Selector/1 -> Discrete Filter/1
  Selector1/1 -> Discrete Filter1/1
  Selector2/1 -> Discrete Filter2/1
  Rate Transition/1 -> Bus Creator/1  "i_conv_dq+"
  Rate Transition1/1 -> Gain1/1, Bus Creator/2  "v_cap_dq+"
  Rate Transition2/1 -> Gain/1, Bus Creator/3  "i_filter_grid_dq+"
  Gain/1 -> Bus Creator/4  "i_grid_dq+"
  Gain1/1 -> Bus Creator/5  "v_grid_dq+"
  theta/1 -> Terminator/1

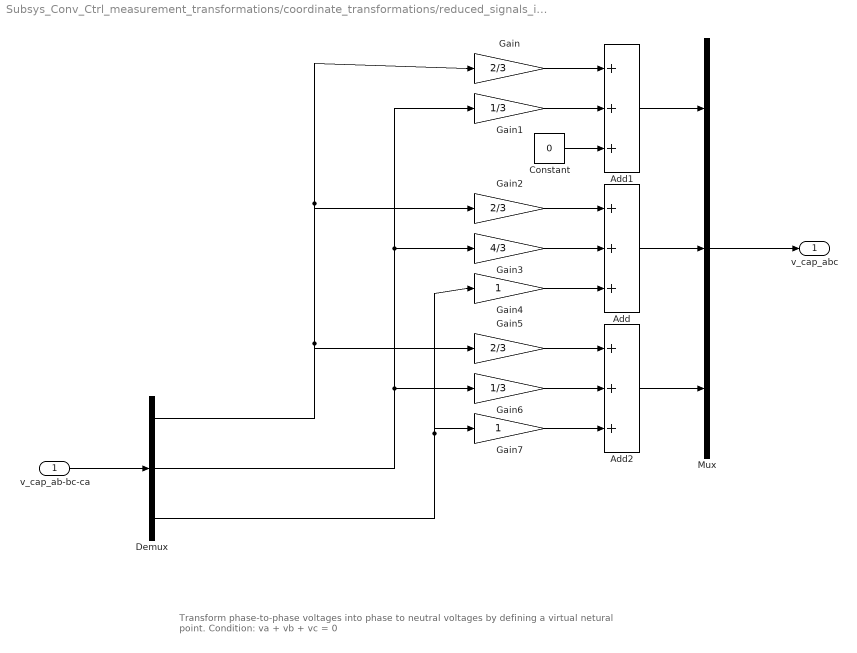
== system Subsys_Conv_Ctrl_measurement_transformations/coordinate_transformations/reduced_signals_imperix_hardware/abc->dq0/DY_transformation ==
  note: Transform phase-to-phase voltages into phase to neutral voltages by defining a virtual netural point. Condition: va + vb + vc = 0
  v_cap_ab-bc-ca : Inport
  Add : Sum  Inputs=+++
  Add1 : Sum  Inputs=+++
  Add2 : Sum  Inputs=+++
  Constant : Constant  Value=0  OutDataTypeStr=datatype
  Demux : Demux  Outputs=3
  Gain : Gain  Gain=2/3
  Gain1 : Gain  Gain=1/3
  Gain2 : Gain  Gain=2/3
  Gain3 : Gain  Gain=4/3
  Gain4 : Gain
  Gain5 : Gain  Gain=2/3
  Gain6 : Gain  Gain=1/3
  Gain7 : Gain
  Mux : Mux  Inputs=3
  v_cap_abc : Outport
  wires:
  v_cap_ab-bc-ca/1 -> Demux/1
  Mux/1 -> v_cap_abc/1
  Add/1 -> Mux/2
  Add1/1 -> Mux/1
  Add2/1 -> Mux/3
  Gain/1 -> Add1/1
  Gain1/1 -> Add1/2
  Constant/1 -> Add1/3
  Gain2/1 -> Add/1
  Gain3/1 -> Add/2
  Gain4/1 -> Add/3
  Gain5/1 -> Add2/1
  Gain6/1 -> Add2/2
  Gain7/1 -> Add2/3
  Demux/1 -> Gain5/1, Gain2/1, Gain/1
  Demux/2 -> Gain6/1, Gain3/1, Gain1/1
  Demux/3 -> Gain7/1, Gain4/1
